simulink model "LKM_Roll_Pitch_AW_Core_Harness"  (R2026b)
settings: Solver=FixedStepDiscrete  StopTime=10  FixedStep=0.01
undefined symbols (not defined in the file): DiscIntNeverNeededParam

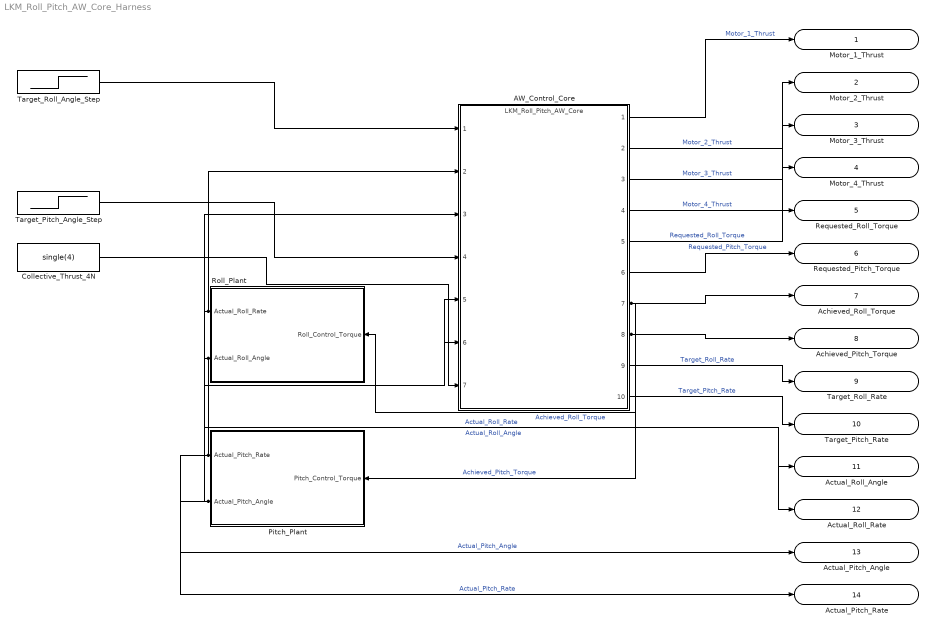
== system LKM_Roll_Pitch_AW_Core_Harness ==
  AW_Control_Core : ModelReference  ModelNameDialog=LKM_Roll_Pitch_AW_Core  SimulationMode=Normal  ModelReferenceVersion=1.1
  Collective_Thrust_4N : Constant  Value=single(4)  OutDataTypeStr=single
  Pitch_Plant : Subsystem
  Roll_Plant : Subsystem
  Target_Pitch_Angle_Step : Step  FinalValue=-3*pi/180  OutDataTypeStr=single  SampleTime=0
  Target_Roll_Angle_Step : Step  FinalValue=5*pi/180  OutDataTypeStr=single  SampleTime=0
  Motor_1_Thrust : Outport
  Motor_2_Thrust : Outport  Port=2
  Motor_3_Thrust : Outport  Port=3
  Motor_4_Thrust : Outport  Port=4
  Requested_Roll_Torque : Outport  Port=5
  Requested_Pitch_Torque : Outport  Port=6
  Achieved_Roll_Torque : Outport  Port=7
  Achieved_Pitch_Torque : Outport  Port=8
  Target_Roll_Rate : Outport  Port=9
  Target_Pitch_Rate : Outport  Port=10
  Actual_Roll_Angle : Outport  Port=11
  Actual_Roll_Rate : Outport  Port=12
  Actual_Pitch_Angle : Outport  Port=13
  Actual_Pitch_Rate : Outport  Port=14
  wires:
  Target_Roll_Angle_Step/1 -> AW_Control_Core/1
  Target_Pitch_Angle_Step/1 -> AW_Control_Core/4
  Collective_Thrust_4N/1 -> AW_Control_Core/7
  Roll_Plant/1(Actual_Roll_Rate) -> AW_Control_Core/2, Actual_Roll_Rate/1  "Actual_Roll_Rate"
  Roll_Plant/2(Actual_Roll_Angle) -> AW_Control_Core/3, Actual_Roll_Angle/1  "Actual_Roll_Angle"
  Pitch_Plant/1(Actual_Pitch_Rate) -> AW_Control_Core/5, Actual_Pitch_Rate/1  "Actual_Pitch_Rate"
  Pitch_Plant/2(Actual_Pitch_Angle) -> AW_Control_Core/6, Actual_Pitch_Angle/1  "Actual_Pitch_Angle"
  AW_Control_Core/7 -> Roll_Plant/1(Roll_Control_Torque), Achieved_Roll_Torque/1  "Achieved_Roll_Torque"
  AW_Control_Core/8 -> Pitch_Plant/1(Pitch_Control_Torque), Achieved_Pitch_Torque/1  "Achieved_Pitch_Torque"
  AW_Control_Core/1 -> Motor_1_Thrust/1  "Motor_1_Thrust"
  AW_Control_Core/2 -> Motor_2_Thrust/1  "Motor_2_Thrust"
  AW_Control_Core/3 -> Motor_3_Thrust/1  "Motor_3_Thrust"
  AW_Control_Core/4 -> Motor_4_Thrust/1  "Motor_4_Thrust"
  AW_Control_Core/5 -> Requested_Roll_Torque/1  "Requested_Roll_Torque"
  AW_Control_Core/6 -> Requested_Pitch_Torque/1  "Requested_Pitch_Torque"
  AW_Control_Core/9 -> Target_Roll_Rate/1  "Target_Roll_Rate"
  AW_Control_Core/10 -> Target_Pitch_Rate/1  "Target_Pitch_Rate"

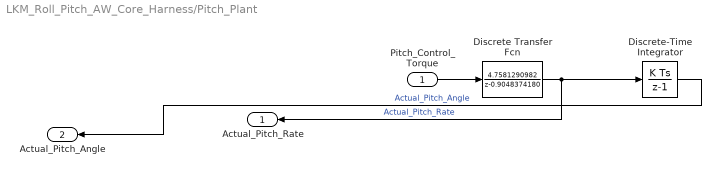
== system LKM_Roll_Pitch_AW_Core_Harness/Pitch_Plant ==
  Pitch_Control_Torque : Inport
  Discrete Transfer Fcn : DiscreteTransferFcn  Numerator=[0 4.7581290982]  Denominator=[1 -0.9048374180]
  Discrete-Time Integrator : DiscreteIntegrator  SampleTime=0.01  ICPrevOutput=DiscIntNeverNeededParam  ICPrevScaledInput=DiscIntNeverNeededParam
  Actual_Pitch_Rate : Outport
  Actual_Pitch_Angle : Outport  Port=2
  wires:
  Discrete-Time Integrator/1 -> Actual_Pitch_Angle/1  "Actual_Pitch_Angle"
  Pitch_Control_Torque/1 -> Discrete Transfer Fcn/1
  Discrete Transfer Fcn/1 -> Discrete-Time Integrator/1, Actual_Pitch_Rate/1  "Actual_Pitch_Rate"

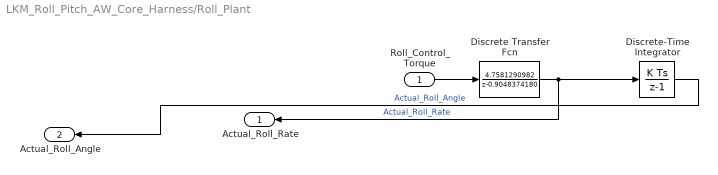
== system LKM_Roll_Pitch_AW_Core_Harness/Roll_Plant ==
  Roll_Control_Torque : Inport
  Discrete Transfer Fcn : DiscreteTransferFcn  Numerator=[0 4.7581290982]  Denominator=[1 -0.9048374180]
  Discrete-Time Integrator : DiscreteIntegrator  SampleTime=0.01  ICPrevOutput=DiscIntNeverNeededParam  ICPrevScaledInput=DiscIntNeverNeededParam
  Actual_Roll_Rate : Outport
  Actual_Roll_Angle : Outport  Port=2
  wires:
  Roll_Control_Torque/1 -> Discrete Transfer Fcn/1
  Discrete Transfer Fcn/1 -> Discrete-Time Integrator/1, Actual_Roll_Rate/1  "Actual_Roll_Rate"
  Discrete-Time Integrator/1 -> Actual_Roll_Angle/1  "Actual_Roll_Angle"
